simulink model "ExplorePath"  (R2025b)
settings: Solver=ode4  StartTime=0.0  StopTime=simulation.stoptime  FixedStep=simulation.sampletime  RelTol=1e-3  EnableMultiTasking=on
values from neighbouring files (symbols this model uses):
  asv = mpsv.designer.ASV()    [Initialize.m]
  K = result.explorePath.matK    [Initialize.m]
  rpsi = min(rpsi, manualLimitRadiusPsi)    [Initialize.m]
  rx = min(rx, manualLimitRadiusX)    [Initialize.m]
  ry = min(ry, manualLimitRadiusY)    [Initialize.m]
undefined symbols (not defined in the file or in its folder): simulation
settings Model: Creator=damerius  LastModifiedBy=damerius
settings SolverCC: ConcurrentTasks=on
settings DataIOCC: SaveOutput=off  SignalLogging=off  DSMLogging=off  SaveTime=off  ReturnWorkspaceOutputs=off
settings OptimizationCC: DefaultParameterBehavior=Inlined  EnhancedBackFolding=on  PassReuseOutputArgsAs=Individual arguments  ZeroExternalMemoryAtStartup=off  ZeroInternalMemoryAtStartup=off  SimCompilerOptimization=on  OptimizeBlockOrder=speed  DifferentSizesBufferReuse=on  OptimizationCustomize=off  EfficientTunableParamExpr=on
settings DebuggingCC: ParameterTunabilityLossMsg=error  UnconnectedInputMsg=warning  UnconnectedOutputMsg=warning  UnconnectedLineMsg=warning
settings HardwareCC: ProdBitPerLong=64.0  ProdHWDeviceType=Intel->x86-64 (Linux 64)  TargetBitPerLong=64.0  TargetBitPerPointer=64.0  TargetBitPerSizeT=64.0  TargetBitPerPtrDiffT=64.0  TargetLargestAtomicFloat=Float  TargetIntDivRoundTo=Zero  TargetEndianess=LittleEndian  TargetWordSize=64.0  TargetHWDeviceType=Intel->x86-64 (Linux 64)  ProdEqTarget=off
settings ModelReferenceCC: EnableRefExpFcnMdlSchedulingChecks=on
settings SFSimCC: SimGenImportedTypeDefs=on  SimTargetLang=C++  SimDLTargetLibrary=mkl-dnn
settings RTWCC: SystemTargetFile=ert.tlc  GenCodeOnly=on  PackageGeneratedCodeAndArtifacts=on  PackageName=PackNGo  TemplateMakefile=ert_default_tmf  Toolchain=CMake  DataTypeReplacement=CDataTypesFixedWidth  TargetLang=C++  Description=Embedded Coder
settings CodeAppCC: ForceParamTrailComments=on  IgnoreCustomStorageClasses=off  MaxIdLength=128.0  OperatorAnnotations=on  SimulinkDataObjDesc=on  SFDataObjDesc=on  InsertBlockDesc=on  StateflowObjectComments=on  MATLABSourceComments=on  UseSimReservedNames=on
settings ERTTargetCC: TargetOS=NativeThreadsExample  RootIOFormat=Structure reference  ERTCustomFileTemplate=example_file_process.tlc  IndentSize=4  NewlineStyle=LF  MaxLineWidth=256.0  MaxIdInt64=INT64_MAX  MinIdInt64=INT64_MIN  MaxIdUint64=UINT64_MAX  MaxIdInt32=INT32_MAX  MinIdInt32=INT32_MIN  MaxIdUint32=UINT32_MAX  MaxIdInt16=INT16_MAX  MinIdInt16=INT16_MIN  MaxIdUint16=UINT16_MAX  MaxIdInt8=INT8_MAX  MinIdInt8=INT8_MIN  MaxIdUint8=UINT8_MAX  DynamicArrayContainerType=coder::array  TargetLangStandard=C++20 (ISO)  CodeInterfacePackaging=C++ class  SubcomponentCodeInterfacePackaging=C++ class  SupportContinuousTime=on  SupportVariableSizeSignals=on

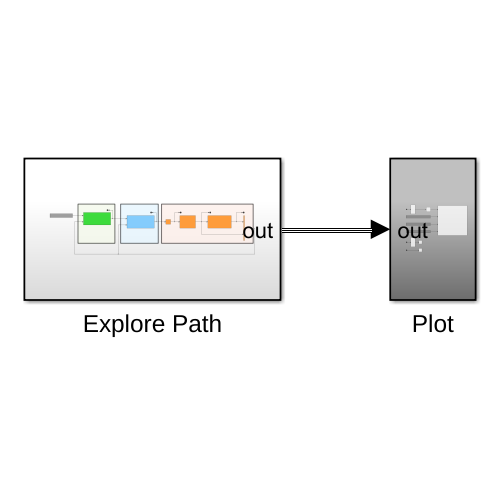
[thumbnail: Simulink's stored preview of the top-level diagram]
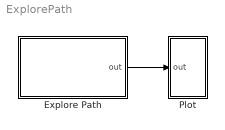
== system ExplorePath ==
  Explore Path : Subsystem
  Plot : Subsystem
  wires:
  Explore Path/1(out) -> Plot/1(out)

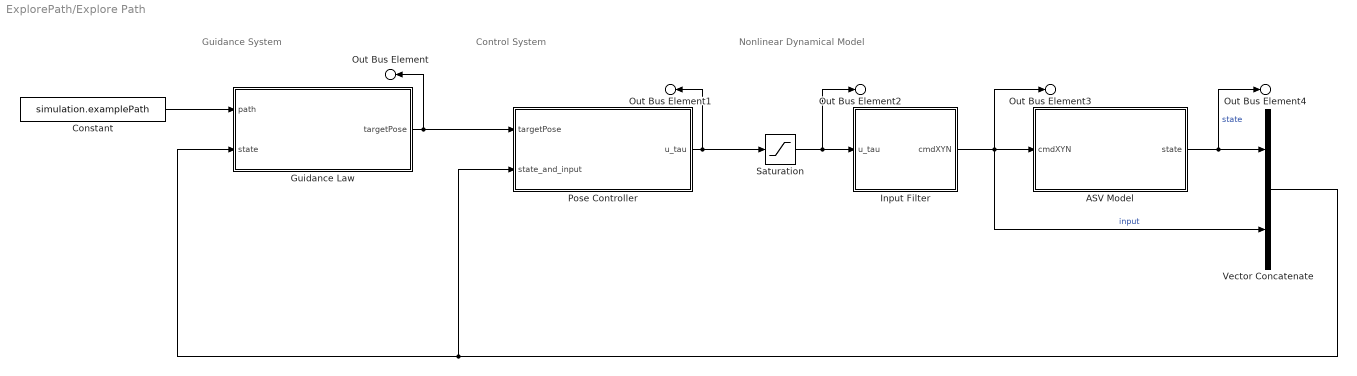
== system ExplorePath/Explore Path ==
  note: Nonlinear Dynamical Model
  note: Control System
  note: Guidance System
  ASV Model : Subsystem
  Constant : Constant  Value=simulation.examplePath
  Guidance Law : Subsystem
  Input Filter : Subsystem
  Pose Controller : Subsystem
  Saturation : Saturate  UpperLimit=asv.model.vecSatXYN  LowerLimit=-asv.model.vecSatXYN
  Vector Concatenate : Concatenate
  Out Bus Element : Outport  PortName=out  Element=targetPose
  Out Bus Element1 : Outport  PortName=out  Element=u_tau
  Out Bus Element2 : Outport  PortName=out  Element=u_tau_sat
  Out Bus Element3 : Outport  PortName=out  Element=cmdXYN
  Out Bus Element4 : Outport  PortName=out  Element=state
  wires:
  Saturation/1 -> Input Filter/1(u_tau), Out Bus Element2/1
  Input Filter/1(cmdXYN) -> Out Bus Element3/1, ASV Model/1(cmdXYN), Vector Concatenate/2  "input"
  Vector Concatenate/1 -> Guidance Law/2(state), Pose Controller/2(state_and_input)
  Constant/1 -> Guidance Law/1(path)
  ASV Model/1(state) -> Out Bus Element4/1, Vector Concatenate/1  "state"
  Guidance Law/1(targetPose) -> Out Bus Element/1, Pose Controller/1(targetPose)
  Pose Controller/1(u_tau) -> Out Bus Element1/1, Saturation/1

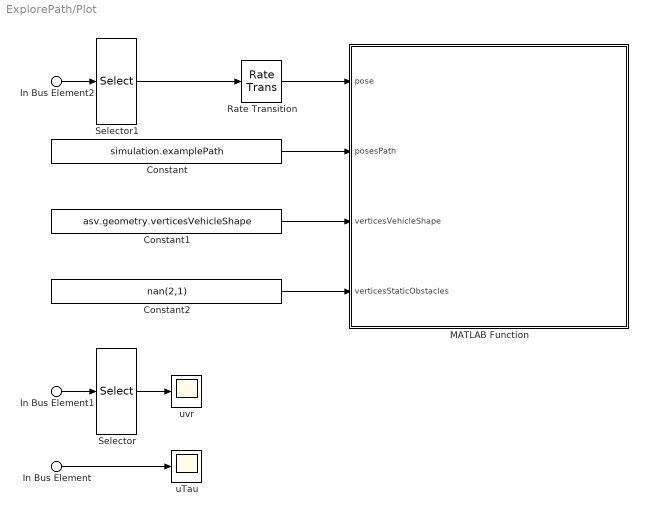
== system ExplorePath/Plot ==
  In Bus Element : Inport  PortName=out  Element=u_tau_sat
  In Bus Element1 : Inport  PortName=out  Element=state
  In Bus Element2 : Inport  PortName=out  Element=state
  Constant : Constant  Value=simulation.examplePath
  Constant1 : Constant  Value=asv.geometry.verticesVehicleShape
  Constant2 : Constant  Value=nan(2,1)
  MATLAB Function : MATLAB Function  TreatAsAtomicUnit=on
  Rate Transition : RateTransition  Deterministic=off  OutPortSampleTime=3
  Selector : Selector  InputPortWidth=9  IndexOptions=Index vector (dialog)  Indices=4:6  OutputSizes=1
  Selector1 : Selector  InputPortWidth=9  IndexOptions=Index vector (dialog)  Indices=1:3  OutputSizes=1
  uTau : Scope
      settings: ActiveDisplayYMinimum=-500  ActiveDisplayYMaximum=500
  uvr : Scope
      settings: ActiveDisplayYMinimum=-1.1985631038102735  ActiveDisplayYMaximum=1.45307497264896
  wires:
  In Bus Element/1 -> uTau/1
  In Bus Element1/1 -> Selector/1
  Selector/1 -> uvr/1
  In Bus Element2/1 -> Selector1/1
  Selector1/1 -> Rate Transition/1
  Rate Transition/1 -> MATLAB Function/1(pose)
  Constant/1 -> MATLAB Function/2(posesPath)
  Constant1/1 -> MATLAB Function/3(verticesVehicleShape)
  Constant2/1 -> MATLAB Function/4(verticesStaticObstacles)

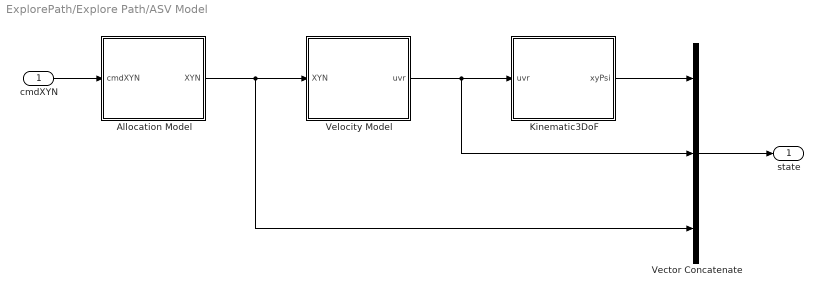
== system ExplorePath/Explore Path/ASV Model ==
  cmdXYN : Inport
  Allocation Model : Subsystem
  Kinematic3DoF : Subsystem
  Vector Concatenate : Concatenate  NumInputs=3
  Velocity Model : Subsystem
  state : Outport
  wires:
  Allocation Model/1(XYN) -> Velocity Model/1(XYN), Vector Concatenate/3
  Vector Concatenate/1 -> state/1
  Velocity Model/1(uvr) -> Vector Concatenate/2, Kinematic3DoF/1(uvr)
  Kinematic3DoF/1(xyPsi) -> Vector Concatenate/1
  cmdXYN/1 -> Allocation Model/1(cmdXYN)

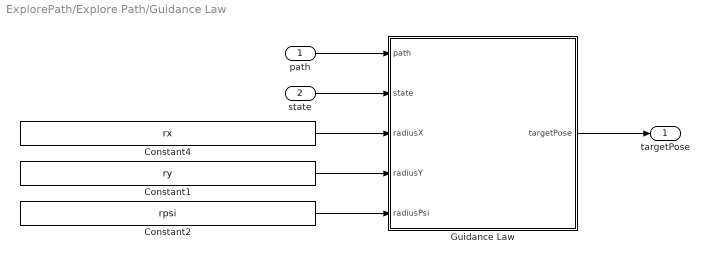
== system ExplorePath/Explore Path/Guidance Law ==
  path : Inport
  state : Inport  Port=2
  Constant1 : Constant  Value=ry
  Constant2 : Constant  Value=rpsi
  Constant4 : Constant  Value=rx
  Guidance Law : MATLAB Function  TreatAsAtomicUnit=on
  targetPose : Outport
  wires:
  path/1 -> Guidance Law/1(path)
  state/1 -> Guidance Law/2(state)
  Guidance Law/1(targetPose) -> targetPose/1
  Constant4/1 -> Guidance Law/3(radiusX)
  Constant1/1 -> Guidance Law/4(radiusY)
  Constant2/1 -> Guidance Law/5(radiusPsi)

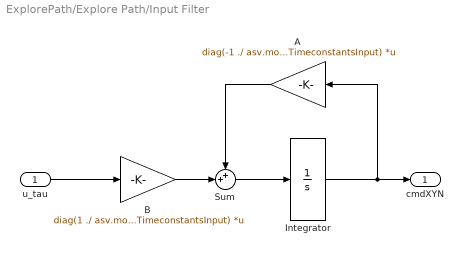
== system ExplorePath/Explore Path/Input Filter ==
  u_tau : Inport
  A : Gain  Gain=diag(-1 ./ asv.model.vecTimeconstantsInput)  Multiplication=Matrix(K*u)
  B : Gain  Gain=diag(1 ./ asv.model.vecTimeconstantsInput)  Multiplication=Matrix(K*u)
  Integrator : Integrator  InitialCondition=[0;0;0]
  Sum : Sum  Inputs=++|
  cmdXYN : Outport
  wires:
  A/1 -> Sum/1
  Integrator/1 -> A/1, cmdXYN/1
  u_tau/1 -> B/1
  Sum/1 -> Integrator/1
  B/1 -> Sum/2

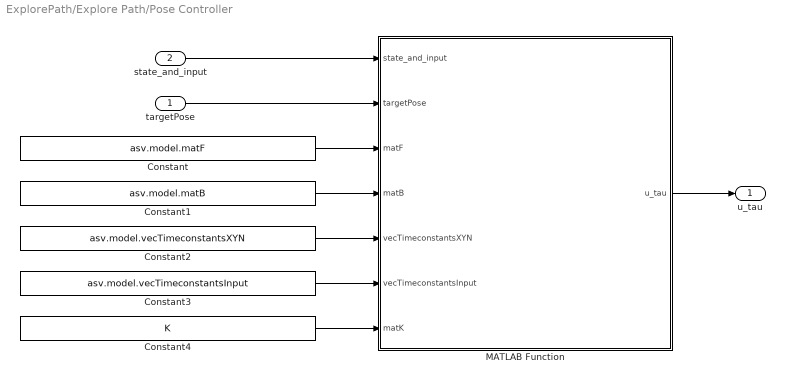
== system ExplorePath/Explore Path/Pose Controller ==
  targetPose : Inport
  state_and_input : Inport  Port=2
  Constant : Constant  Value=asv.model.matF
  Constant1 : Constant  Value=asv.model.matB
  Constant2 : Constant  Value=asv.model.vecTimeconstantsXYN
  Constant3 : Constant  Value=asv.model.vecTimeconstantsInput
  Constant4 : Constant  Value=K
  MATLAB Function : MATLAB Function  TreatAsAtomicUnit=on
  u_tau : Outport
  wires:
  Constant3/1 -> MATLAB Function/6(vecTimeconstantsInput)
  Constant2/1 -> MATLAB Function/5(vecTimeconstantsXYN)
  Constant/1 -> MATLAB Function/3(matF)
  Constant4/1 -> MATLAB Function/7(matK)
  state_and_input/1 -> MATLAB Function/1(state_and_input)
  Constant1/1 -> MATLAB Function/4(matB)
  MATLAB Function/1(u_tau) -> u_tau/1
  targetPose/1 -> MATLAB Function/2(targetPose)

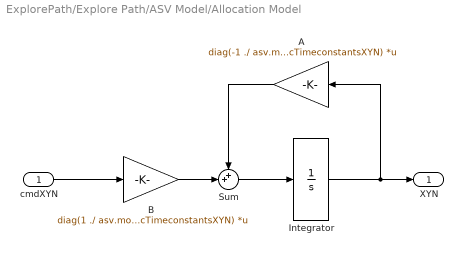
== system ExplorePath/Explore Path/ASV Model/Allocation Model ==
  cmdXYN : Inport
  A : Gain  Gain=diag(-1 ./ asv.model.vecTimeconstantsXYN)  Multiplication=Matrix(K*u)
  B : Gain  Gain=diag(1 ./ asv.model.vecTimeconstantsXYN)  Multiplication=Matrix(K*u)
  Integrator : Integrator  InitialCondition=[0;0;0]
  Sum : Sum  Inputs=++|
  XYN : Outport
  wires:
  B/1 -> Sum/2
  Sum/1 -> Integrator/1
  cmdXYN/1 -> B/1
  Integrator/1 -> XYN/1, A/1
  A/1 -> Sum/1

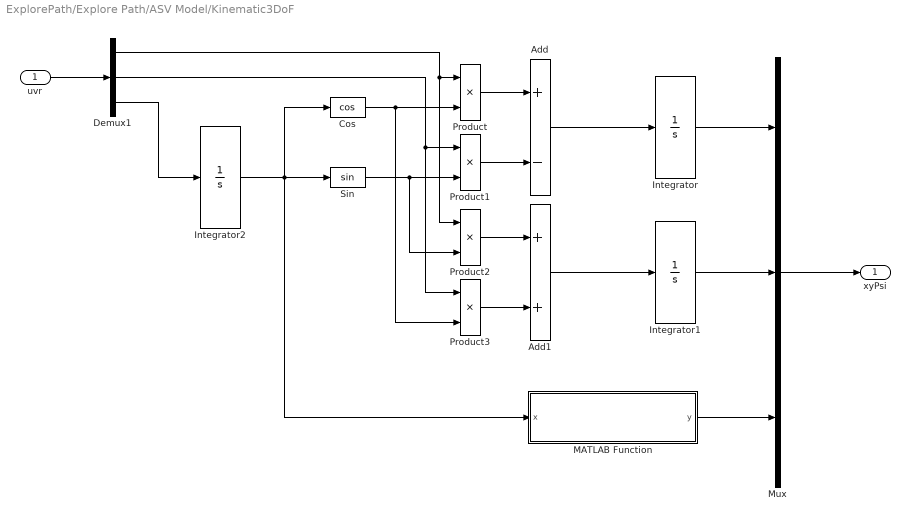
== system ExplorePath/Explore Path/ASV Model/Kinematic3DoF ==
  uvr : Inport  OutDataTypeStr=double  PortDimensions=3
  Add : Sum  Inputs=+-
  Add1 : Sum
  Cos : Trigonometry  Operator=cos
  Demux1 : Demux  Outputs=3
  Integrator : Integrator
  Integrator1 : Integrator
  Integrator2 : Integrator
  MATLAB Function : MATLAB Function  TreatAsAtomicUnit=on
  Mux : Mux  Inputs=3
  Product{,1..3} (4 alike) : Product
  Sin : Trigonometry
  xyPsi : Outport  OutDataTypeStr=double  PortDimensions=3
  wires:
  Mux/1 -> xyPsi/1
  MATLAB Function/1(y) -> Mux/3
  Integrator/1 -> Mux/1
  Integrator1/1 -> Mux/2
  Demux1/3 -> Integrator2/1
  uvr/1 -> Demux1/1
  Add1/1 -> Integrator1/1
  Demux1/1 -> Product/1, Product2/1
  Product/1 -> Add/1
  Add/1 -> Integrator/1
  Product1/1 -> Add/2
  Product3/1 -> Add1/2
  Cos/1 -> Product3/2, Product/2
  Integrator2/1 -> Sin/1, Cos/1, MATLAB Function/1(x)
  Demux1/2 -> Product1/1, Product3/1
  Sin/1 -> Product2/2, Product1/2
  Product2/1 -> Add1/1

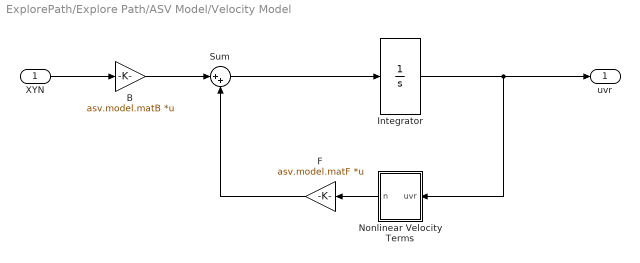
== system ExplorePath/Explore Path/ASV Model/Velocity Model ==
  XYN : Inport
  B : Gain  Gain=asv.model.matB  Multiplication=Matrix(K*u)
  F : Gain  Gain=asv.model.matF  Multiplication=Matrix(K*u)
  Integrator : Integrator  InitialCondition=[0;0;0]
  Nonlinear Velocity Terms : Subsystem
  Sum : Sum  Inputs=|++
  uvr : Outport
  wires:
  F/1 -> Sum/2
  Integrator/1 -> Nonlinear Velocity Terms/1(uvr), uvr/1
  XYN/1 -> B/1
  B/1 -> Sum/1
  Sum/1 -> Integrator/1
  Nonlinear Velocity Terms/1(n) -> F/1

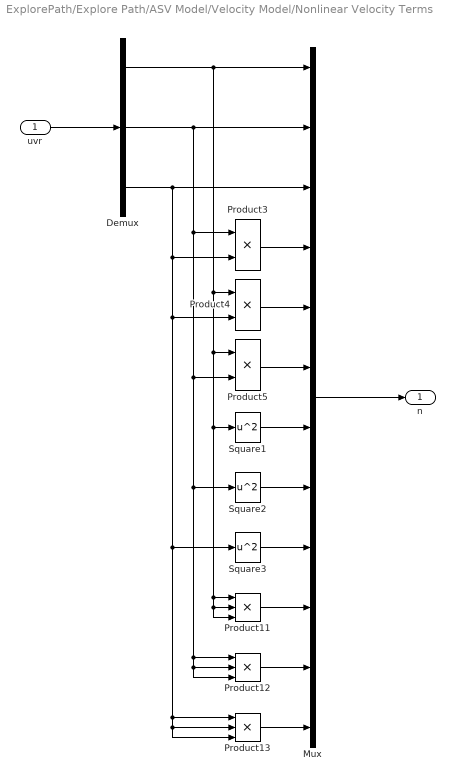
== system ExplorePath/Explore Path/ASV Model/Velocity Model/Nonlinear Velocity Terms ==
  uvr : Inport
  Demux : Demux  Outputs=3
  Mux : Mux  Inputs=12
  Product11 : Product  Inputs=3
  Product12 : Product  Inputs=3
  Product13 : Product  Inputs=3
  Product3 : Product
  Product4 : Product
  Product5 : Product
  Square1 : Math  Operator=square
  Square2 : Math  Operator=square
  Square3 : Math  Operator=square
  n : Outport
  wires:
  uvr/1 -> Demux/1
  Product13/1 -> Mux/12
  Product12/1 -> Mux/11
  Product11/1 -> Mux/10
  Square1/1 -> Mux/7
  Product5/1 -> Mux/6
  Product4/1 -> Mux/5
  Product3/1 -> Mux/4
  Demux/2 -> Product3/1, Product5/2, Square2/1, Product12/1, Product12/3, Product12/2, Mux/2
  Demux/3 -> Product3/2, Product4/2, Square3/1, Product13/1, Product13/3, Product13/2, Mux/3
  Demux/1 -> Mux/1, Product4/1, Product5/1, Square1/1, Product11/1, Product11/3, Product11/2
  Mux/1 -> n/1
  Square2/1 -> Mux/8
  Square3/1 -> Mux/9

== matlab function ExplorePath/Explore Path/ASV Model/Kinematic3DoF/MATLAB Function ==
  data: x input; y output
function y = SymmetricalAngle(x)
    pi2 = pi + pi;
    x = x - pi2 * fix(x / pi2);
    y = x + pi2 * (double(x < -pi) - double(x >= pi));
end

== matlab function ExplorePath/Explore Path/Pose Controller/MATLAB Function ==
  data: state_and_input input; targetPose input; u_tau output; matF input; matB input; vecTimeconstantsXYN input; vecTimeconstantsInput input; matK input
function u_tau = NonlinearPoseControl(state_and_input, targetPose, matF, matB, vecTimeconstantsXYN, vecTimeconstantsInput, matK)
    % ~~~~~~~~~~~~~~~~~~~~~~~~~~~~~~~~~~~~~~~~~~~~~~~~~~~~~~~~~~~~~~
    % Precalculate parameters
    % ~~~~~~~~~~~~~~~~~~~~~~~~~~~~~~~~~~~~~~~~~~~~~~~~~~~~~~~~~~~~~~
    invBBB = diag(vecTimeconstantsXYN .* vecTimeconstantsInput) / matB;
    M0 = -matB ./ vecTimeconstantsXYN;
    f17_2 = 2.0 * matF(1,7);
    f18_2 = 2.0 * matF(1,8);
    f19_2 = 2.0 * matF(1,9);
    f1a_3 = 3.0 * matF(1,10);
    f1b_3 = 3.0 * matF(1,11);
    f1c_3 = 3.0 * matF(1,12);
    f27_2 = 2.0 * matF(2,7);
    f28_2 = 2.0 * matF(2,8);
    f29_2 = 2.0 * matF(2,9);
    f2a_3 = 3.0 * matF(2,10);
    f2b_3 = 3.0 * matF(2,11);
    f2c_3 = 3.0 * matF(2,12);
    f37_2 = 2.0 * matF(3,7);
    f38_2 = 2.0 * matF(3,8);
    f39_2 = 2.0 * matF(3,9);
    f3a_3 = 3.0 * matF(3,10);
    f3b_3 = 3.0 * matF(3,11);
    f3c_3 = 3.0 * matF(3,12);
    f1a_6 = 6.0 * matF(1,10);
    f1b_6 = 6.0 * matF(1,11);
    f1c_6 = 6.0 * matF(1,12);
    f2a_6 = 6.0 * matF(2,10);
    f2b_6 = 6.0 * matF(2,11);
    f2c_6 = 6.0 * matF(2,12);
    f3a_6 = 6.0 * matF(3,10);
    f3b_6 = 6.0 * matF(3,11);
    f3c_6 = 6.0 * matF(3,12);

    % current state and input
    x = state_and_input(1);
    y = state_and_input(2);
    psi = state_and_input(3);
    u = state_and_input(4);
    v = state_and_input(5);
    r = state_and_input(6);
    X = state_and_input(7);
    Y = state_and_input(8);
    N = state_and_input(9);
    Xc = state_and_input(10);
    Yc = state_and_input(11);
    Nc = state_and_input(12);


    % ~~~~~~~~~~~~~~~~~~~~~~~~~~~~~~~~~~~~~~~~~~~~~~~~~~~~~~~~~~~~~~
    % Feedback linearization: calculate useful model terms and compensation
    % ~~~~~~~~~~~~~~~~~~~~~~~~~~~~~~~~~~~~~~~~~~~~~~~~~~~~~~~~~~~~~~
    % forced response velocity model: f(nu) = F*n(nu) + B*tau, where n(nu) = (u,v,r,v*r,u*r,u*v,u^2,v^2,r^2,u^3,v^3,r^3)^T
    forcedResponse = matF * [u; v; r; v*r; u*r; u*v; u*u; v*v; r*r; u*u*u; v*v*v; r*r*r] + matB * [X; Y; N];

    % forced response allocation model: A_tau * tau + B_tau * tau_c
    allocationModel = [Xc - X; Yc - Y; Nc - N] ./ vecTimeconstantsXYN;

    % Jacobian J = df(nu)/dnu (uvr model w.r.t. uvr)
    J = matF(1:3,1:3) + [
        matF(1,5)*r + matF(1,6)*v + f17_2*u + f1a_3*u*u, matF(1,4)*r + matF(1,6)*u + f18_2*v + f1b_3*v*v, matF(1,4)*v + matF(1,5)*u + f19_2*r + f1c_3*r*r;
        matF(2,5)*r + matF(2,6)*v + f27_2*u + f2a_3*u*u, matF(2,4)*r + matF(2,6)*u + f28_2*v + f2b_3*v*v, matF(2,4)*v + matF(2,5)*u + f29_2*r + f2c_3*r*r;
        matF(3,5)*r + matF(3,6)*v + f37_2*u + f3a_3*u*u, matF(3,4)*r + matF(3,6)*u + f38_2*v + f3b_3*v*v, matF(3,4)*v + matF(3,5)*u + f39_2*r + f3c_3*r*r
    ];

    % S0 matrix: J^2 + T, where t_m1 = (dj_m1/du, dj_m2/du, dj_m2/du)*forcedResponse, t_m2 = (dj_m1/dv, dj_m2/dv, dj_m2/dv)*forcedResponse, t_m3 = (dj_m1/dr, dj_m2/dr, dj_m2/dr)*forcedResponse for m=1,2,3
    S0 = J*J + [
        (f17_2 + f1a_6*u)*forcedResponse(1) + matF(1,6)*forcedResponse(2) + matF(1,5)*forcedResponse(3), matF(1,6)*forcedResponse(1) + (f18_2 + f1b_6*v)*forcedResponse(2) + matF(1,4)*forcedResponse(3), matF(1,5)*forcedResponse(1) + matF(1,4)*forcedResponse(2) + (f19_2 + f1c_6*r)*forcedResponse(3);
        (f27_2 + f2a_6*u)*forcedResponse(1) + matF(2,6)*forcedResponse(2) + matF(2,5)*forcedResponse(3), matF(2,6)*forcedResponse(1) + (f28_2 + f2b_6*v)*forcedResponse(2) + matF(2,4)*forcedResponse(3), matF(2,5)*forcedResponse(1) + matF(2,4)*forcedResponse(2) + (f29_2 + f2c_6*r)*forcedResponse(3);
        (f37_2 + f3a_6*u)*forcedResponse(1) + matF(3,6)*forcedResponse(2) + matF(3,5)*forcedResponse(3), matF(3,6)*forcedResponse(1) + (f38_2 + f3b_6*v)*forcedResponse(2) + matF(3,4)*forcedResponse(3), matF(3,5)*forcedResponse(1) + matF(3,4)*forcedResponse(2) + (f39_2 + f3c_6*r)*forcedResponse(3)
    ];

    % S1 matrix: J * B
    S1 = J * matB;

    % flat state vector
    z = [u; v; r; forcedResponse; J * forcedResponse + matB * allocationModel];
 
    % compensation = S0(uvr) * forcedResponse + S1(uvr) * allocationModel + M0 * (allocationModel + Bc*tau_c)
    tmp = allocationModel + [Xc; Yc; Nc] ./ vecTimeconstantsInput;
    compensation = S0 * forcedResponse + S1 * allocationModel + M0 * tmp;


    % ~~~~~~~~~~~~~~~~~~~~~~~~~~~~~~~~~~~~~~~~~~~~~~~~~~~~~~~~~~~~~~
    % Pose controller (flat state controller with respect to target pose as origin)
    % ~~~~~~~~~~~~~~~~~~~~~~~~~~~~~~~~~~~~~~~~~~~~~~~~~~~~~~~~~~~~~~
    dx = x - targetPose(1);
    dy = y - targetPose(2);
    c = cos(psi);
    s = sin(psi);
    deltaPose = [c*dx + s*dy; -s*dx + c*dy; SymmetricalAngle(psi - targetPose(3))];

    % Calculate the flat state control command using the control law uz = -K * [deltaPose; z1; z2; z3]
    uz = -matK * [deltaPose; z];

    % final control law uTau = invBBB * (uz - compensation)
    u_tau = invBBB * (uz - compensation);
end

function y = SymmetricalAngle(x)
    pi2 = pi + pi;
    x = x - pi2 * fix(x / pi2);
    y = x + pi2 * (double(x < -pi) - double(x >= pi));
end

== matlab function ExplorePath/Plot/MATLAB Function ==
  data: pose input; posesPath input; verticesVehicleShape input; verticesStaticObstacles input
function FigureDisplay(pose, posesPath, verticesVehicleShape, verticesStaticObstacles)
    persistent f;
    if(isempty(f))
        f = figure(42);
    end
    persistent posesHistory;
    if(isempty(posesHistory))
        posesHistory = pose;
    else
        posesHistory = [posesHistory, pose];
    end

    clf;
    hold on;
    PlotPath(posesPath, verticesVehicleShape, [0 0.3 0.5]);
    PlotPath(posesHistory, verticesVehicleShape, [0.9 0 0]);
    PlotObstacles(verticesStaticObstacles);
    view(90,-90);
    axis equal;
    box on;
    grid on;
    xlabel('x in m');
    ylabel('y in m');
    title('Explore Path');
    drawnow();
end

function PlotPath(poses, verticesVehicleShape, color)
    numPoses = size(poses, 2);
    x = poses(1,1:numPoses);
    y = poses(2,1:numPoses);
    plot(x,y,'LineWidth',2,'Color',color);
    for i = uint32(1):uint32(numPoses)
        PlotVehicleShape(poses(:,i), verticesVehicleShape, color);
    end
end

function PlotVehicleShape(pose, verticesVehicleShape, color)
    c = cos(pose(3));
    s = sin(pose(3));
    R = [c -s; s c];

    N = int32(size(verticesVehicleShape,2));
    i0 = int32(-1);

    for i = int32(1):N
        finiteVertex = isfinite(verticesVehicleShape(1,i)) && isfinite(verticesVehicleShape(2,i));
        if((i0 < 1) && finiteVertex)
            i0 = i;
        elseif((i0 > 0) && (~finiteVertex || (i == N)))
            i = i + int32((i == N) && finiteVertex);
            vertices = R * verticesVehicleShape(:,i0:(i-1)) + [pose(1); pose(2)];
            PlotPolygon(vertices, color);
            plot(pose(1),pose(2),'o','Color',color);
            i0 = int32(-1);
        end
    end
end

function PlotObstacles(verticesStaticObstacles)
    N = int32(size(verticesStaticObstacles,2));
    i0 = int32(-1);

    for i = int32(1):N
        finiteVertex = isfinite(verticesStaticObstacles(1,i)) && isfinite(verticesStaticObstacles(2,i));
        if((i0 < 1) && finiteVertex)
            i0 = i;
        elseif((i0 > 0) && (~finiteVertex || (i == N)))
            i = i + int32((i == N) && finiteVertex);
            PlotPolygon(verticesStaticObstacles(:,i0:(i-1)), [0,0,0]);
            i0 = int32(-1);
        end
    end
end

function PlotPolygon(vertices, color)
    x = [vertices(1,:) vertices(1,1)];
    y = [vertices(2,:) vertices(2,1)];
    plot(x,y,'LineWidth',1,'Color',color);
end

== matlab function ExplorePath/Explore Path/Guidance Law/Guidance Law ==
  data: path input; state input; radiusX input; radiusY input; radiusPsi input; targetPose output
function targetPose = GuidanceLaw(path, state, radiusX, radiusY, radiusPsi)
    invSquaredRadiusX = 1.0 / (radiusX * radiusX);
    invSquaredRadiusY = 1.0 / (radiusY * radiusY);
    invSquaredRadiusPsi = 1.0 / (radiusPsi * radiusPsi);
    pose = state(1:3);
    targetPose = PathGuidance(pose, path, invSquaredRadiusX, invSquaredRadiusY, invSquaredRadiusPsi);
end

function targetPose = PathGuidance(pose, path, invSquaredRadiusX, invSquaredRadiusY, invSquaredRadiusPsi)
    % The path guidance law calculates a target pose based on a given path and the current pose of the vehicle. The target pose
    % corresponds to the intersection point of the path with an ellipsoid, which is located at the pose of the vehicle. The major
    % and minor axes of that ellipsoid point in the longitudinal and lateral direction of the vehicles body frame. The dimension
    % of the ellpsoid is set by three radii - a longitudinal radius (X), a lateral radius (Y) and a radius for the heading angle
    % (Psi). This function requires the inverse of the squareroot of the corresponding radii, that is 1/(R*R).
    % 
    % - If the ellipsoid intersects the path at several points, then that point being closest to the end of the path along that
    %   path is used.
    % 
    % - If there's no intersection point of the path with that ellipsoid, then the closest point of the ellipsoid to the path is
    %   used as target pose. This function thus ensures, that the distance between the given pose and the resulting target pose is
    %   not larger than the specified radii of the ellipsoid.
    % 
    % - If the final pose of the path is within the ellipsoid, then this final pose is used as target pose.
    % 
    % - If the specified path is empty, then the current vehicle pose is used as target pose.
    %
    % - If the path consists of only one pose, then the line from the vehicles pose to that single pose is used as path to find
    %   the intersection with the ellipsoid.
    % 
    % 
    % PARAMETER
    % pose                 ... 3-by-1 vector: Input pose that denotes the current vehicle pose, given as [x; y; psi].
    % path                 ... 3-by-N matrix: Input path desribed by a list of poses. Each pose is given as [x; y; psi].
    % invSquaredRadiusX    ... 1 / r^2 with r being the radius for the longitudinal distance (b-frame) for the waypoint guidance law.
    % invSquaredRadiusY    ... 1 / r^2 with r being the radius for the lateral distance (b-frame) for the waypoint guidance law.
    % invSquaredRadiusPsi  ... 1 / r^2 with r being the radius for the angular distance for the waypoint guidance law.
    % 
    % RESULT
    % targetPose ... Output target pose, given as [x; y; psi].
    assert((3 == size(pose,1)) && (1 == size(pose,2)));
    assert((3 == size(path,1)));

    % To find the intersection point of an rotated ellipsoid with a path in SE(2), the path is transformed into a corresponding
    % euclidean space R^3, whose origin is located at the vehicles pose. The space transformation is done in such a way, that
    % the intersection simplifies to finding the intersection of a line in 3D space with a 3D unit sphere centered at the
    % vehicles pose. For a given vehicle pose [x; y; psi] any pose of the path [x_i; y_i; psi_i] can be transformed into the
    % euclidean space by
    % 
    %    ( p_ix )   (1/rx  0    0    )   ( cos(psi)  sin(psi)  0)   (     x_i - x   )
    %    ( p_iy ) = ( 0   1/ry  0    ) * (-sin(psi)  cos(psi)  0) * (     y_i - y   )
    %    (p_ipsi)   ( 0    0   1/rpsi)   (    0         0      1)   (SA(psi_i - psi))  ,
    % 
    % where rx,ry,rpsi denote the radii for longitudinal, lateral and angular direction, respectively, and SA() denotes the
    % symmetrical angle function. Assume, the path is given by five points [q0, q1, q2, q3, q4] and the vehicle pose is given by
    % eta = [x;y;psi].
    % 
    %    q0                 q1                 q2                 q3                 q4
    %     o ---------------- o ---------------- o ---------------- o ---------------- o
    % 
    % 
    % 
    %                                o eta
    % 
    % 
    % All poses of the path are transformed into the euclidean space and eta denotes the origin of that space. The guidance law
    % consists of two main steps.
    % 
    % 
    % STEP 1: FIND CLOSEST INTERPOLATED POSE
    % In the first step the closest interapolated pose along the path is searched for.
    % 
    %                             closest interpolated pose (pI)
    %                                |
    %     p0                p1       V         p2                 p3                 p4
    %      o - - - - - - - - o - - - x -------- o ---------------- o ---------------- o
    %                                :
    %                                :
    %                                :
    %                                o origin [0;0;0]
    % 
    % Now the actual path of interest consists of the origin, the closest interpolated pose and p2, p3, p4. This path
    % [0, pI, p2, p3, p4] always intersects with a unit sphere around the origin.
    % 
    % 
    % STEP 2: FIND FIRST INTERSECTION
    % In the second step, it is iterated through all line segments, starting from the origin. The first line segment that
    % intersects with the unit sphere, gives the commanded pose in the transformed euclidean space. The intersection point is
    % defined by the equation
    % 
    %  pc = pa + lambda * (pb - pa)  ,
    % 
    % where pa and pb denote two consecutive points, e.g. starting and ending point of a specific line segment. If a lambda is
    % found, then the corresponding intersection pose is calculated by the same equation but in SE(2).
    % 
    % eta_c = SA(eta_a + lambda * SA(eta_b - eta_a))  ,
    % 
    % where SA() ensures, that the angular dimension is handled correctly and remains in [-pi, +pi).
    % 
    %                                    intersection point (target point pc)
    %                                                  |
    %       p0              p1      pI         p2      V         p3                 p4
    %        o   -   -   -   o   -   o -------- o -----x---------- o ---------------- o
    %                                :                  ' 
    %                                :                   ' 
    %                                :                    :
    %                                o <~~~~~~~~~~~~~~~~> :
    %                                        r = 1        :
    %                                                    ,
    %                                                   ,
    % 
    % If the end of the path is within the unit sphere, e.g. |p4| < 1, then pc is equal to p4.

    % Some variables and constants
    pa = [0;0;0];
    pb = [0;0;0];
    cpsi = cos(pose(3));
    spsi = sin(pose(3));
    numWaypoints = size(path, 2);

    % The fallback value if the path is empty
    targetPose = pose;
    if(numWaypoints < 1)
        return;
    end

    % STEP 1: Get the closest interpolated pose on the path to the given pose
    idxSegment = [0;0]; % stores the indices (zero-based) of the start and end point from a line segment
    interpolation = 0.0; % stores the lambda value (interpolation ratio) for that line segment
    if(numWaypoints > 1)
        % Go through all line segments and search for the lowest squared distance
        lowestSquaredDistance = inf;

        % Initial starting point pa for first segment (pa without 1/r scale)
        dx = path(1,1) - pose(1);
        dy = path(2,1) - pose(2);
        pa(1) = cpsi * dx + spsi * dy;
        pa(2) = -spsi * dx + cpsi * dy;
        pa(3) = SymmetricalAngle(path(3,1) - pose(3));
        for n = 1:(numWaypoints-1) % n: zero-based index
            % For each line segment: calculate the interpolation factor lambda that minimizes the distance from pose to the current line segment
            % Starting point pa is already given, calculate ending point pb for this line segment (also without 1/r scale)
            dx = path(1,n+1) - pose(1);
            dy = path(2,n+1) - pose(2);
            pb(1) = cpsi * dx + spsi * dy;
            pb(2) = -spsi * dx + cpsi * dy;
            pb(3) = SymmetricalAngle(path(3,n+1) - pose(3));

            % Calculate lambda of p = pa + lambda*(pb - pa), where p is closest to the origin (here we consider the neglected 1/r scale)
            % lambda = (pa' * (pa - pb) / ((pa - pb)' * (pa - pb)))
            dx = pa(1) - pb(1);
            dy = pa(2) - pb(2);
            dz = pa(3) - pb(3);
            denominator = invSquaredRadiusX*dx*dx + invSquaredRadiusY*dy*dy + invSquaredRadiusPsi*dz*dz;
            lambda = 0.0;
            if(abs(denominator) > eps())
                lambda = (invSquaredRadiusX*pa(1)*dx + invSquaredRadiusY*pa(2)*dy + invSquaredRadiusPsi*pa(3)*dz) / denominator;
            end

            % Clamp lambda to line segment [0, 1]
            lambda = min(max(lambda,0.0),1.0);

            % Calculate squared distance from pI = [sx; sy; sz] from origin in transformed R3 space and check if distance is reduced
            sx = pa(1) - lambda * dx;
            sy = pa(2) - lambda * dy;
            sz = pa(3) - lambda * dz;
            squaredDistance = invSquaredRadiusX*sx*sx + invSquaredRadiusY*sy*sy + invSquaredRadiusPsi*sz*sz;
            if(squaredDistance < lowestSquaredDistance)
                lowestSquaredDistance = squaredDistance;
                idxSegment(1) = n - 1;
                idxSegment(2) = n;
                interpolation = lambda;
            end

            % Set the ending point of this line segment as starting point for the next line segment
            pa = pb;
        end
    end
    interpolatedPose = [0;0;0];
    interpolatedPose(1) = path(1,idxSegment(1)+1) + interpolation * (path(1,idxSegment(2)+1) - path(1,idxSegment(1)+1));
    interpolatedPose(2) = path(2,idxSegment(1)+1) + interpolation * (path(2,idxSegment(2)+1) - path(2,idxSegment(1)+1));
    interpolatedPose(3) = SymmetricalAngle(path(3,idxSegment(1)+1) + interpolation * SymmetricalAngle(path(3,idxSegment(2)+1) - path(3,idxSegment(1)+1)));

    % STEP 2: Find the target pose, that is, the intersection of the ellipsoid with the path.
    % The path to be considered starts from the given pose and continues with the closest interpolated pose followed by all remaining poses
    % from the input path. The order is: pose --> interpolatedPose --> path[idxSegment[1]] --> ... --> path[end]. Because this path starts
    % at the pose, there's always an intersection of the ellipsoid with the line segment if the length of the linesegment is non-zero.

    % Line segment 1: pose --> interpolatedPose
    % We set pa to the interpolated pose (without 1/r scale) because this is the starting point for the next line segment
    dx = interpolatedPose(1) - pose(1);
    dy = interpolatedPose(2) - pose(2);
    pa(1) = cpsi * dx + spsi * dy;
    pa(2) = -spsi * dx + cpsi * dy;
    pa(3) = SymmetricalAngle(interpolatedPose(3) - pose(3));
    L = invSquaredRadiusX*pa(1)*pa(1) + invSquaredRadiusY*pa(2)*pa(2) + invSquaredRadiusPsi*pa(3)*pa(3); % take into account 1/r scale
    if(L > 1.0)
        lambda = 1.0 / sqrt(L);
        targetPose(1) = pose(1) + lambda * dx;
        targetPose(2) = pose(2) + lambda * dy;
        targetPose(3) = SymmetricalAngle(pose(3) + lambda * pa(3));
        return;
    end
    targetPose = interpolatedPose;

    % Line segment 2: interpolatedPose --> path[idxSegment[1]]
    % pa is already known from line segment 1, calculate end point pb (also without 1/r scale)
    dx = path(1,idxSegment(2)+1) - pose(1);
    dy = path(2,idxSegment(2)+1) - pose(2);
    pb(1) = cpsi * dx + spsi * dy;
    pb(2) = -spsi * dx + cpsi * dy;
    pb(3) = SymmetricalAngle(path(3,idxSegment(2)+1) - pose(3));
    dx = pb(1) - pa(1);
    dy = pb(2) - pa(2);
    dz = pb(3) - pa(3);
    a = invSquaredRadiusX*dx*dx + invSquaredRadiusY*dy*dy + invSquaredRadiusPsi*dz*dz;
    bHalf = (invSquaredRadiusX*pa(1)*dx + invSquaredRadiusY*pa(2)*dy + invSquaredRadiusPsi*pa(3)*dz);
    c = invSquaredRadiusX*pa(1)*pa(1) + invSquaredRadiusY*pa(2)*pa(2) + invSquaredRadiusPsi*pa(3)*pa(3) - 1.0;
    if(a > eps())
        sr = sqrt(bHalf * bHalf - a * c);
        lambda = max((-bHalf + sr) / a, (-bHalf - sr) / a);
        if(lambda <= 1.0)
            targetPose(1) = interpolatedPose(1) + lambda * (path(1,idxSegment(2)+1) - interpolatedPose(1));
            targetPose(2) = interpolatedPose(2) + lambda * (path(2,idxSegment(2)+1) - interpolatedPose(2));
            targetPose(3) = SymmetricalAngle(interpolatedPose(3) + lambda * SymmetricalAngle(path(3,idxSegment(2)+1) - interpolatedPose(3)));
            return;
        end
    end
    targetPose = path(:,idxSegment(2)+1);

    % Line segments 3,...: path[idxSegment[1]] --> ... --> path[end]
    for i = (idxSegment(2)+1):(numWaypoints-1) % zero-based index
        % Start point pa is previous end point pb
        pa = pb;

        % Calculate the endpoint of this line segment (again without 1/r scale)
        dx = path(1,i+1) - pose(1);
        dy = path(2,i+1) - pose(2);
        pb(1) = cpsi * dx + spsi * dy;
        pb(2) = -spsi * dx + cpsi * dy;
        pb(3) = SymmetricalAngle(path(3,i+1) - pose(3));
        dx = pb(1) - pa(1);
        dy = pb(2) - pa(2);
        dz = pb(3) - pa(3);
        a = invSquaredRadiusX*dx*dx + invSquaredRadiusY*dy*dy + invSquaredRadiusPsi*dz*dz;
        bHalf = (invSquaredRadiusX*pa(1)*dx + invSquaredRadiusY*pa(2)*dy + invSquaredRadiusPsi*pa(3)*dz);
        c = invSquaredRadiusX*pa(1)*pa(1) + invSquaredRadiusY*pa(2)*pa(2) + invSquaredRadiusPsi*pa(3)*pa(3) - 1.0;
        if(a > eps())
            sr = sqrt(bHalf * bHalf - a * c);
            lambda = max((-bHalf + sr) / a, (-bHalf - sr) / a);
            if(lambda <= 1.0)
                targetPose(1) = path(1,i) + lambda * (path(1,i+1) - path(1,i));
                targetPose(2) = path(2,i) + lambda * (path(2,i+1) - path(2,i));
                targetPose(3) = SymmetricalAngle(path(3,i) + lambda * SymmetricalAngle(path(3,i+1) - path(3,i)));
                return;
            end
        end
        targetPose = path(:,i+1);
    end
    targetPose(3) = SymmetricalAngle(targetPose(3));
end

function y = SymmetricalAngle(x)
    pi2 = pi + pi;
    x = x - pi2 * fix(x / pi2);
    y = x + pi2 * (double(x < -pi) - double(x >= pi));
end
